simulink model "Projectile_friction_and_ground_modeling"  (R2023b)
settings: Solver=FixedStepAuto  StartTime=0.0  StopTime=duree_simu  FixedStep=1/10  RelTol=1e-3
values from neighbouring files (symbols this model uses):
  coef_frottement = 0.04    [Projectile_parameters.m]
  gravite = 9.81    [Projectile_parameters.m]
  masse = 15    [Projectile_parameters.m]
  pos_x0 = 0    [Projectile_parameters.m]    (also in parametres_TP_projectile.m)
  pos_y0 = 0    [Projectile_parameters.m]    (also in parametres_TP_projectile.m)
  vit_x0 = vit0*cos(theta)    [Projectile_parameters.m]    (also in parametres_TP_projectile.m)
  vit_y0 = vit0*sin(theta)    [Projectile_parameters.m]    (also in parametres_TP_projectile.m)
libraries: simulink x2
settings Model: Creator=Moi  LastModifiedBy=T0144666
settings SolverCC: AlgebraicLoopSolver=TrustRegion
settings DataIOCC: ReturnWorkspaceOutputs=off
settings OptimizationCC: ReuseModelBlockBuffer=off
settings DebuggingCC: UnconnectedInputMsg=warning  UnconnectedOutputMsg=warning  UnconnectedLineMsg=warning  ArithmeticOperatorsInVariantConditions=warning
settings ModelReferenceCC: EnableRefExpFcnMdlSchedulingChecks=on
settings SFSimCC: SimUseLocalCustomCode=off  CustomCodeUndefinedFunction=UseInterfaceOnly
settings RTWCC: RTWUseLocalCustomCode=off  DLArmComputeVersion=19.05

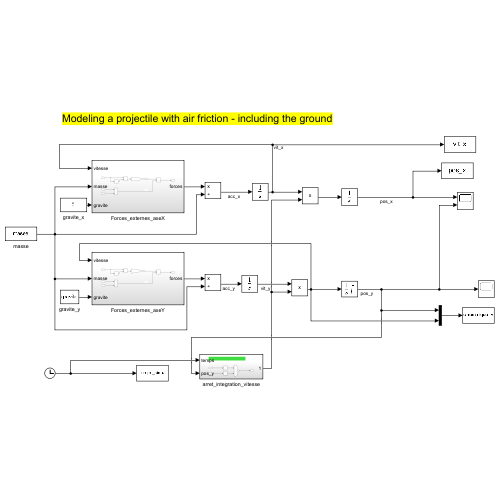
[thumbnail: Simulink's stored preview of the top-level diagram]
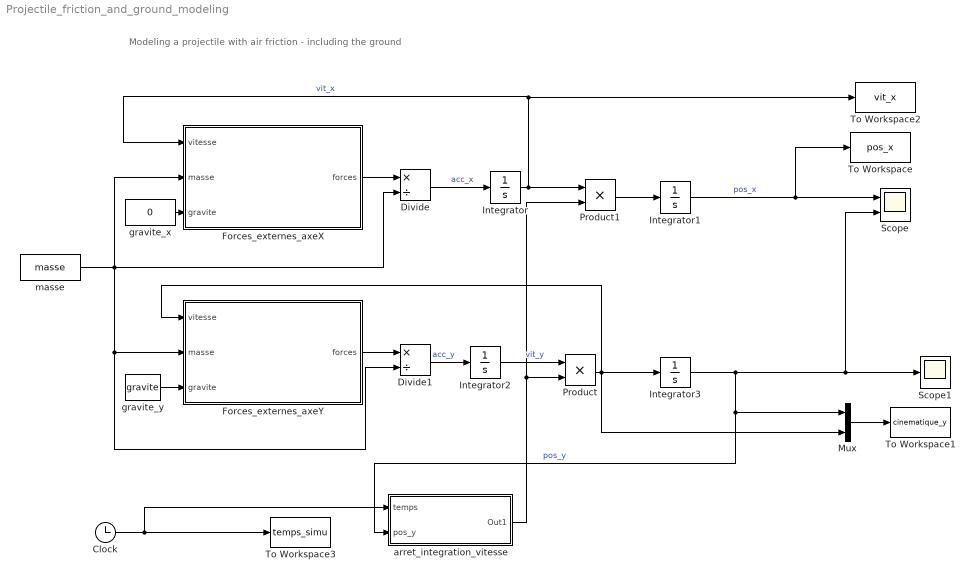
== system Projectile_friction_and_ground_modeling ==
  note: Modeling a projectile with air friction - including the ground
  Clock : Clock
  Divide : Product  Inputs=*/
  Divide1 : Product  Inputs=*/
  Forces_externes_axeX : Subsystem
  Forces_externes_axeY : Subsystem
  Integrator : Integrator  InitialCondition=vit_x0
  Integrator1 : Integrator  InitialCondition=pos_x0
  Integrator2 : Integrator  InitialCondition=vit_y0
  Integrator3 : Integrator  InitialCondition=pos_y0  LimitOutput=on  LowerSaturationLimit=0
  Mux : Mux  Inputs=2
  Product : Product
  Product1 : Product
  Scope : Scope  NumInputPorts=2
  Scope1 : Scope
  To Workspace : ToWorkspace  VariableName=pos_x  SampleTime=-1
  To Workspace1 : ToWorkspace  VariableName=cinematique_y  SampleTime=-1
  To Workspace2 : ToWorkspace  VariableName=vit_x  SampleTime=-1
  To Workspace3 : ToWorkspace  VariableName=temps_simu  SampleTime=-1
  arret_integration_vitesse : Subsystem
  gravite_x : Constant  Value=0
  gravite_y : Constant  Value=gravite
  masse : Constant  Value=masse
  wires:
  masse/1 -> Forces_externes_axeX/2(masse), Divide/2, Divide1/2, Forces_externes_axeY/2(masse)
  gravite_x/1 -> Forces_externes_axeX/3(gravite)
  Forces_externes_axeX/1(forces) -> Divide/1
  Integrator/1 -> Forces_externes_axeX/1(vitesse), To Workspace2/1, Product1/1  "vit_x"
  Divide/1 -> Integrator/1  "acc_x"
  Integrator1/1 -> To Workspace/1, Scope/1  "pos_x"
  gravite_y/1 -> Forces_externes_axeY/3(gravite)
  Forces_externes_axeY/1(forces) -> Divide1/1
  Divide1/1 -> Integrator2/1  "acc_y"
  Mux/1 -> To Workspace1/1
  Clock/1 -> arret_integration_vitesse/1(temps), To Workspace3/1
  Integrator3/1 -> arret_integration_vitesse/2(pos_y), Mux/1, Scope/2, Scope1/1  "pos_y"
  Integrator2/1 -> Product/1  "vit_y"
  Product/1 -> Mux/2, Forces_externes_axeY/1(vitesse), Integrator3/1
  Product1/1 -> Integrator1/1
  arret_integration_vitesse/1(Out1) -> Product1/2, Product/2

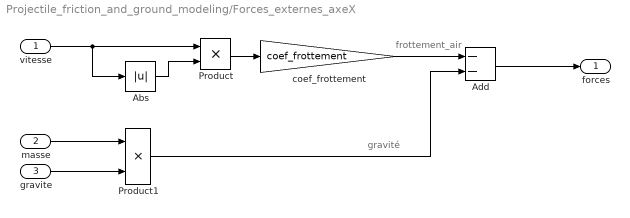
== system Projectile_friction_and_ground_modeling/Forces_externes_axeX ==
  note: frottement_air
  note: gravité
  vitesse : Inport
  masse : Inport  Port=2
  gravite : Inport  Port=3
  Abs : Abs  SaturateOnIntegerOverflow=off
  Add : Sum  Inputs=--
  Product : Product
  Product1 : Product
  coef_frottement : Gain  Gain=coef_frottement
  forces : Outport  VectorParamsAs1DForOutWhenUnconnected=off
  wires:
  Product/1 -> coef_frottement/1
  masse/1 -> Product1/1
  coef_frottement/1 -> Add/1
  Abs/1 -> Product/2
  gravite/1 -> Product1/2
  Product1/1 -> Add/2
  vitesse/1 -> Abs/1, Product/1
  Add/1 -> forces/1

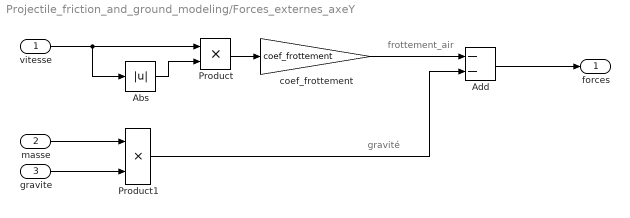
== system Projectile_friction_and_ground_modeling/Forces_externes_axeY ==
  note: frottement_air
  note: gravité
  vitesse : Inport
  masse : Inport  Port=2
  gravite : Inport  Port=3
  Abs : Abs  SaturateOnIntegerOverflow=off
  Add : Sum  Inputs=--
  Product : Product
  Product1 : Product
  coef_frottement : Gain  Gain=coef_frottement
  forces : Outport  VectorParamsAs1DForOutWhenUnconnected=off
  wires:
  Product/1 -> coef_frottement/1
  masse/1 -> Product1/1
  coef_frottement/1 -> Add/1
  gravite/1 -> Product1/2
  Product1/1 -> Add/2
  vitesse/1 -> Abs/1, Product/1
  Add/1 -> forces/1
  Abs/1 -> Product/2

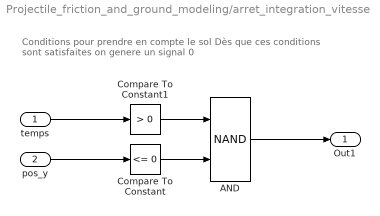
== system Projectile_friction_and_ground_modeling/arret_integration_vitesse ==
  note: Conditions pour prendre en compte le sol
      | Dès que ces conditions sont satisfaites on genere un signal 0
  temps : Inport
  pos_y : Inport  Port=2
  AND : Logic  Operator=NAND  IconShape=distinctive  AllPortsSameDT=off  OutDataTypeStr=boolean
  Compare To Constant : simulink/Logic and Bit Operations/Compare To Constant  relop=<=  const=0  OutDataTypeStr=boolean
  Compare To Constant1 : simulink/Logic and Bit Operations/Compare To Constant  relop=>  const=0  OutDataTypeStr=boolean
  Out1 : Outport
  wires:
  Compare To Constant1/1 -> AND/1
  pos_y/1 -> Compare To Constant/1
  Compare To Constant/1 -> AND/2
  AND/1 -> Out1/1
  temps/1 -> Compare To Constant1/1
